simulink library "flexibleBody_lib"  (R2018b)
settings: Solver=VariableStepAuto  StartTime=0.0  StopTime=10.0  RelTol=1e-3
undefined symbols (not defined in the file or in its folder): structure, structure_red, structureGetNodeCg, structureGetNodeMass, structureGetTotalInertia, structureGetTotalMass
libraries: rigidBody_lib x1
settings Model: Creator=Ybeyer  LastModifiedBy=yannic
settings DebuggingCC: LibraryContextMissingDiagnostic=none
settings SFSimCC: SimUseLocalCustomCode=off
settings RTWCC: RTWUseLocalCustomCode=off
settings CodeAppCC: StateflowObjectComments=on

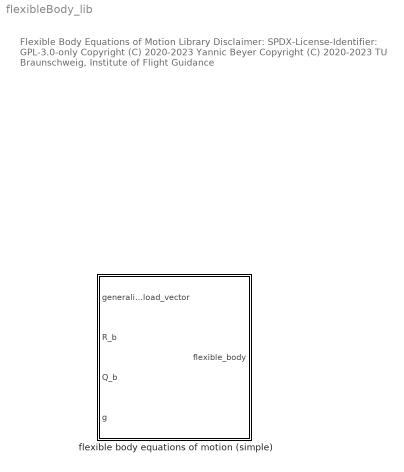
== system flexibleBody_lib ==
  note: Flexible Body Equations of Motion Library
      |
      | Disclaimer:
      | SPDX-License-Identifier: GPL-3.0-only
      |
      | Copyright (C) 2020-2023 Yannic Beyer
      | Copyright (C) 2020-2023 TU Braunschweig, Institute of Flight Guidance
  flexible body equations of motion (simple) : Subsystem  mask{structure_red=structure_red, m=structureGetTotalMass(structure), I_b=structureGetTotalInertia(structure), m_nodes=structureGetNodeMass(structure,1:length(structure.xyz)), cg_nodes=structureGetNodeCg(structure,1:length(structure.xyz)), structure_vel_0=zeros(size(structure_red.K,2)-6,1), structure_pos_0=zeros(size(structure_red.K,2)-6,1)}
      mask prompts: structure_red "reduced-order structure struct (see structureGetReduced)"; m "total mass (scalar), in kg"; I_b "total inertia matrix (3x3 array), in kg*m^2"; m_nodes "node masses, in kg"; cg_nodes "node cg position offsets, in m"; structure_vel_0 "initial generalized velocity vector"; structure_pos_0 "initial generalized position vector"
      mask DialogControl DescGroupVar Prompt: Flexible body equations of motion
      mask DialogControl DescTextVar Prompt: Simple implementation according to Waszak and Schmidt.
      mask DialogControl Control3 Prompt: More info can be found in the function documentation inside or in the README:
      mask DialogControl Control4 Prompt: README
      mask DialogControl Control4 Callback: web('https://github.com/iff-gsc/LADAC/blob/main/equations_of_motion/flexible_body_simple/README.md','-browser')

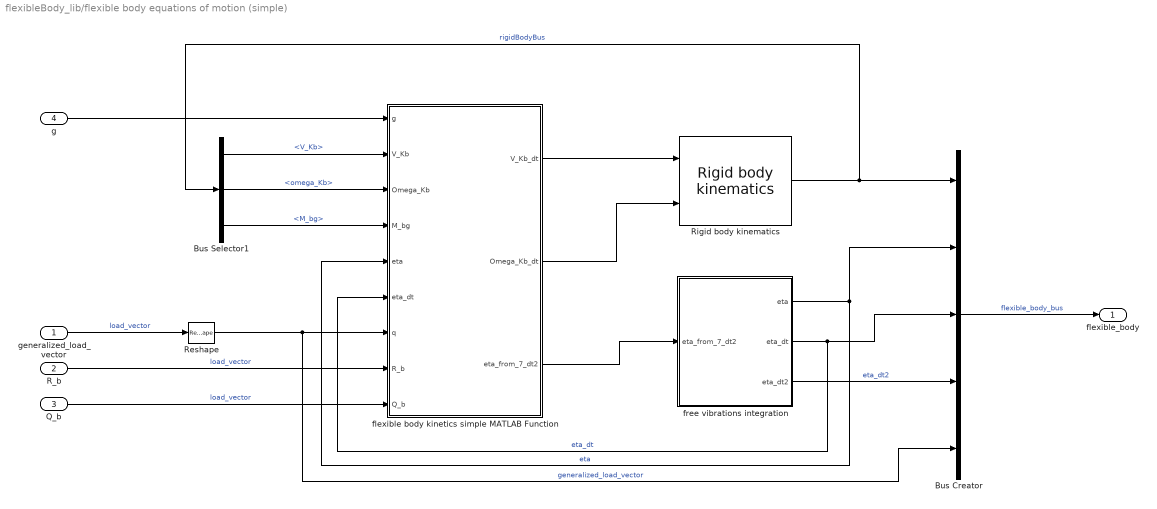
== system flexibleBody_lib/flexible body equations of motion (simple) ==
  generalized_load_vector : Inport
  R_b : Inport  Port=2
  Q_b : Inport  Port=3
  g : Inport  Port=4
  Bus Creator : BusCreator  Inputs=5
  Bus Selector1 : BusSelector  OutputSignals=V_Kb,omega_Kb,M_bg
  Reshape : Reshape  OutputDimensionality=Column vector (2-D)
  Rigid body kinematics : rigidBody_lib/Rigid body kinematics  omega_Kb_0=ic.omega_Kb  q_bg_0=ic.q_bg  V_Kb_0=ic.V_Kb  s_g_0=ic.s_Kg
      settings: SourceProductName=LADAC
  flexible body kinetics simple MATLAB Function : MATLAB Function  TreatAsAtomicUnit=on
  free vibrations integration : Subsystem
  flexible_body : Outport
  wires:
  flexible body kinetics simple MATLAB Function/3(eta_from_7_dt2) -> free vibrations integration/1(eta_from_7_dt2)
  flexible body kinetics simple MATLAB Function/2(Omega_Kb_dt) -> Rigid body kinematics/2
  Bus Creator/1 -> flexible_body/1  "flexible_body_bus"
  Bus Selector1/3 -> flexible body kinetics simple MATLAB Function/4(M_bg)  "<M_bg>"
  free vibrations integration/1(eta) -> Bus Creator/2, flexible body kinetics simple MATLAB Function/5(eta)  "eta"
  Rigid body kinematics/1 -> Bus Selector1/1, Bus Creator/1  "rigidBodyBus"
  Bus Selector1/1 -> flexible body kinetics simple MATLAB Function/2(V_Kb)  "<V_Kb>"
  free vibrations integration/3(eta_dt2) -> Bus Creator/4  "eta_dt2"
  g/1 -> flexible body kinetics simple MATLAB Function/1(g)
  flexible body kinetics simple MATLAB Function/1(V_Kb_dt) -> Rigid body kinematics/1
  generalized_load_vector/1 -> Reshape/1  "load_vector"
  Bus Selector1/2 -> flexible body kinetics simple MATLAB Function/3(Omega_Kb)  "<omega_Kb>"
  free vibrations integration/2(eta_dt) -> flexible body kinetics simple MATLAB Function/6(eta_dt), Bus Creator/3  "eta_dt"
  Reshape/1 -> flexible body kinetics simple MATLAB Function/7(q), Bus Creator/5  "generalized_load_vector"
  R_b/1 -> flexible body kinetics simple MATLAB Function/8(R_b)  "load_vector"
  Q_b/1 -> flexible body kinetics simple MATLAB Function/9(Q_b)  "load_vector"

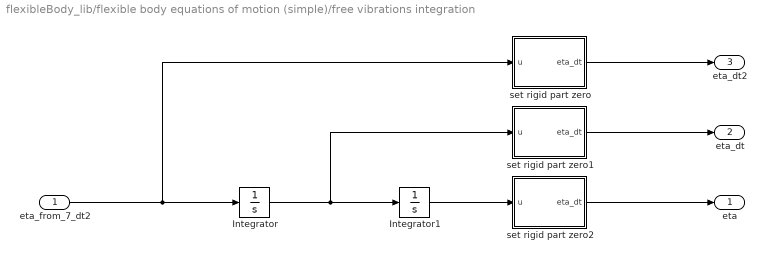
== system flexibleBody_lib/flexible body equations of motion (simple)/free vibrations integration ==
  eta_from_7_dt2 : Inport
  Integrator : Integrator  InitialCondition=structure_vel_0
  Integrator1 : Integrator  InitialCondition=structure_pos_0
  set rigid part zero : MATLAB Function  TreatAsAtomicUnit=on
  set rigid part zero1 : MATLAB Function  TreatAsAtomicUnit=on
  set rigid part zero2 : MATLAB Function  TreatAsAtomicUnit=on
  eta : Outport
  eta_dt : Outport  Port=2
  eta_dt2 : Outport  Port=3
  wires:
  Integrator/1 -> set rigid part zero1/1(u), Integrator1/1
  Integrator1/1 -> set rigid part zero2/1(u)
  eta_from_7_dt2/1 -> set rigid part zero/1(u), Integrator/1
  set rigid part zero/1(eta_dt) -> eta_dt2/1
  set rigid part zero2/1(eta_dt) -> eta/1
  set rigid part zero1/1(eta_dt) -> eta_dt/1

== matlab function flexibleBody_lib/flexible body equations of motion (simple)/free vibrations integration/set rigid part zero1 ==
  data: u input; eta_dt output
function eta_dt = fcn(u) %#codegen
eta_dt = [zeros(6,1);u];
end

== matlab function flexibleBody_lib/flexible body equations of motion (simple)/flexible body kinetics simple MATLAB Function ==
  data: m parameter; I_b parameter; V_Kb_dt output; Omega_Kb_dt output; g input; structure_red parameter; m_nodes parameter; V_Kb input; Omega_Kb input; M_bg input; eta input; eta_dt input; q input; eta_from_7_dt2 output; R_b input; Q_b input; cg_nodes parameter
function [V_Kb_dt,Omega_Kb_dt,eta_from_7_dt2] = ...
    flexibleBodyKineticsSimple( m, I_b, g, structure_red, m_nodes, ...
    V_Kb, Omega_Kb, M_bg, eta, eta_dt, q, R_b, Q_b, cg_nodes)
[V_Kb_dt,Omega_Kb_dt,eta_from_7_dt2] = ...
    flexibleBodyKineticsSimple( m, I_b, g, structure_red, m_nodes, ...
    cg_nodes, V_Kb, Omega_Kb, M_bg, eta, eta_dt, q, R_b, Q_b );
end

== matlab function flexibleBody_lib/flexible body equations of motion (simple)/free vibrations integration/set rigid part zero2 ==
  data: u input; eta_dt output
function eta_dt = fcn(u) %#codegen
eta_dt = [zeros(6,1);u];
end

== matlab function flexibleBody_lib/flexible body equations of motion (simple)/free vibrations integration/set rigid part zero ==
  data: u input; eta_dt output
function eta_dt = fcn(u) %#codegen
eta_dt = [zeros(6,1);u];
end
